simulink model "parcial_2_simulaciones copy"  (R2026b)
settings: Solver=VariableStepAuto  StopTime=20
undefined symbols (not defined in the file): A_LIN, B_LIN, C_LIN, D_LIN, X_INIT
libraries: mpclib x4
settings Model: Creator=santi  LastModifiedBy=ivanm
settings SimscapeCC: SimscapeLogType=all  SimscapeNominalValues="[{\"value\":\"1\",\"unit\":\"A\"},{\"value\":\"1\",\"unit\":\"bar\"},{\"value\":\"1\",\"unit\":\"cm^2\"},{\"value\":\"1\",\"unit\":\"cm^3/s\"},{\"value\":\"1\",\"unit\":\"kJ/kg\"},{\"value\":\"1\",\"unit\":\"kW\"},{\"value\":\"1\",\"unit\":\"l\"},{\"value\":\"1\",\"unit\":\"N\"},{\"value\":\"1\",\"unit\":\"N*m\"},{\"value\":\"1\",\"unit\":\"V\"},{\"value\":\"0.001\",\"unit\":\"Wb\"}]"  SimscapeUseEnergyAccounting=off

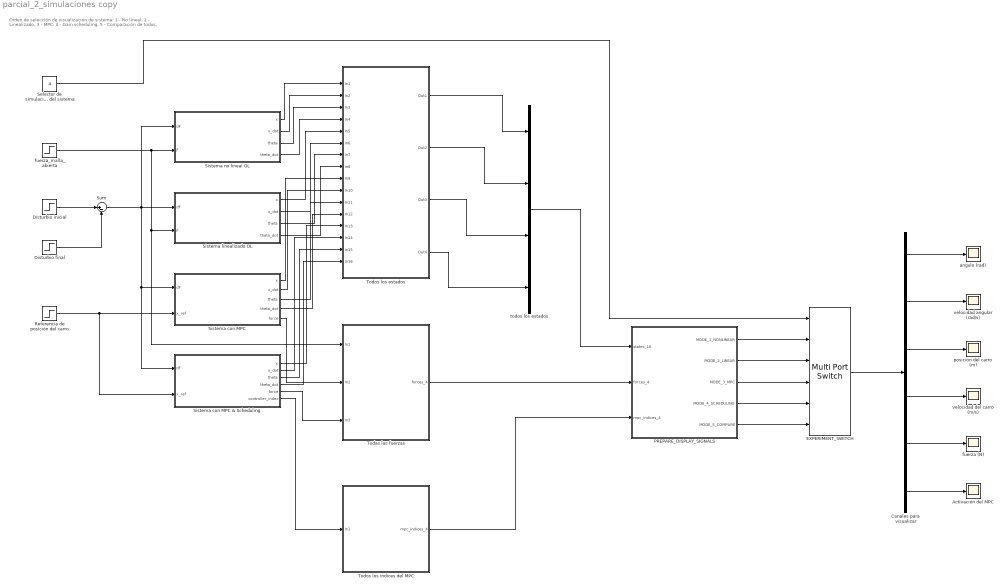
== system parcial_2_simulaciones copy ==
  note: Orden de selección de visualización de sistema:
      |
      | 1 - No lineal.
      | 2 -  Linealizado.
      | 3 - MPC.
      | 4 - Gain scheduling.
      | 5 - Comparación de todos.
  Activación del MPC : Scope
      settings: ActiveDisplayYMinimum=1  ActiveDisplayYMaximum=3  DataLoggingVariableName=ScopeData5
  Canales para visualizar : Demux  Outputs=[4 4 4 4 4 4]
  Disturbio final : Step  Time=4.1  FinalValue=0.05  SampleTime=0
  Disturbio inicial : Step  Time=4  FinalValue=0.05  SampleTime=0
  EXPERIMENT_SWITCH : MultiPortSwitch  Inputs=5  SaturateOnIntegerOverflow=off  InputSameDT=off
  PREPARE_DISPLAY_SIGNALS : Subsystem
  Referencia de posición del carro : Step  FinalValue=0.1  SampleTime=0
  Selector de simulación del sistema : Constant  Value=4
  Sistema con MPC : Subsystem
  Sistema con MPC & Scheduling : Subsystem
  Sistema linealizado OL : Subsystem
  Sistema no lineal OL : Subsystem
  Sum : Sum  Inputs=|+-
  Todas las fuerzas : Subsystem
  Todos los estados : Subsystem
  Todos los indices del MPC : Subsystem
  angulo (rad) : Scope
      settings: ActiveDisplayYMinimum=-0.0688727030292263  ActiveDisplayYMaximum=0.11906082395866187
  fuerza (N) : Scope
      settings: ActiveDisplayYMinimum=-1.8144592130461565  ActiveDisplayYMaximum=0.971895002005476  DataLoggingVariableName=ScopeData4
  fuerza_malla_abierta : Step  Time=0.5  FinalValue=0.05  SampleTime=0
  posición del carro (m) : Scope
      settings: ActiveDisplayYMinimum=-0.040524237311587434  ActiveDisplayYMaximum=0.062688605845198017  DataLoggingVariableName=ScopeData2
  todos los estados : Mux
  velocidad angular (rad/s) : Scope
      settings: ActiveDisplayYMinimum=-0.30702774847885805  ActiveDisplayYMaximum=0.1053556961511582
  velocidad del carro (m/s) : Scope
      settings: ActiveDisplayYMinimum=-0.55827066909262324  ActiveDisplayYMaximum=0.15487434647916765  DataLoggingVariableName=ScopeData3
  wires:
  fuerza_malla_abierta/1 -> Todas las fuerzas/1(In1), Sistema linealizado OL/2(F), Sistema no lineal OL/2(F)
  Disturbio inicial/1 -> Sum/1
  Disturbio final/1 -> Sum/2
  Sum/1 -> Sistema no lineal OL/1(dF), Sistema con MPC/1(dF), Sistema con MPC & Scheduling/1(dF), Sistema linealizado OL/1(dF)
  Referencia de posición del carro/1 -> Sistema con MPC & Scheduling/2(x_ref), Sistema con MPC/2(x_ref)
  Sistema no lineal OL/1(x) -> Todos los estados/1(In1)
  Sistema no lineal OL/2(x_dot) -> Todos los estados/2(In2)
  Sistema no lineal OL/3(theta) -> Todos los estados/3(In3)
  Sistema no lineal OL/4(theta_dot) -> Todos los estados/4(In4)
  Sistema linealizado OL/1(x) -> Todos los estados/5(In5)
  Sistema linealizado OL/2(x_dot) -> Todos los estados/6(In6)
  Sistema linealizado OL/3(theta) -> Todos los estados/7(In7)
  Sistema linealizado OL/4(theta_dot) -> Todos los estados/8(In8)
  Sistema con MPC/1(x) -> Todos los estados/9(In9)
  Sistema con MPC/2(x_dot) -> Todos los estados/10(In10)
  Sistema con MPC/3(theta) -> Todos los estados/11(In11)
  Sistema con MPC/4(theta_dot) -> Todos los estados/12(In12)
  Sistema con MPC & Scheduling/1(x) -> Todos los estados/13(In13)
  Sistema con MPC & Scheduling/2(x_dot) -> Todos los estados/14(In14)
  Sistema con MPC & Scheduling/3(theta) -> Todos los estados/15(In15)
  Sistema con MPC & Scheduling/4(theta_dot) -> Todos los estados/16(In16)
  Sistema con MPC/5(force) -> Todas las fuerzas/2(In2)
  Sistema con MPC & Scheduling/5(force) -> Todas las fuerzas/3(In3)
  Sistema con MPC & Scheduling/6(controller_index) -> Todos los indices del MPC/1(In1)
  PREPARE_DISPLAY_SIGNALS/3(MODE_3_MPC) -> EXPERIMENT_SWITCH/4
  PREPARE_DISPLAY_SIGNALS/4(MODE_4_SCHEDULING) -> EXPERIMENT_SWITCH/5
  PREPARE_DISPLAY_SIGNALS/1(MODE_1_NONLINEAR) -> EXPERIMENT_SWITCH/2
  PREPARE_DISPLAY_SIGNALS/5(MODE_5_COMPARE) -> EXPERIMENT_SWITCH/6
  Todos los estados/1(Out1) -> todos los estados/1
  Todos los estados/2(Out2) -> todos los estados/2
  Todos los estados/3(Out3) -> todos los estados/3
  Todos los estados/4(Out4) -> todos los estados/4
  todos los estados/1 -> PREPARE_DISPLAY_SIGNALS/1(states_16)
  Todas las fuerzas/1(forces_4) -> PREPARE_DISPLAY_SIGNALS/2(forces_4)
  Todos los indices del MPC/1(mpc_indices_4) -> PREPARE_DISPLAY_SIGNALS/3(mpc_indices_4)
  Selector de simulación del sistema/1 -> EXPERIMENT_SWITCH/1
  EXPERIMENT_SWITCH/1 -> Canales para visualizar/1
  Canales para visualizar/1 -> angulo (rad)/1
  Canales para visualizar/2 -> velocidad angular (rad/s)/1
  Canales para visualizar/3 -> posición del carro (m)/1
  Canales para visualizar/4 -> velocidad del carro (m/s)/1
  Canales para visualizar/5 -> fuerza (N)/1
  Canales para visualizar/6 -> Activación del MPC/1
  PREPARE_DISPLAY_SIGNALS/2(MODE_2_LINEAR) -> EXPERIMENT_SWITCH/3

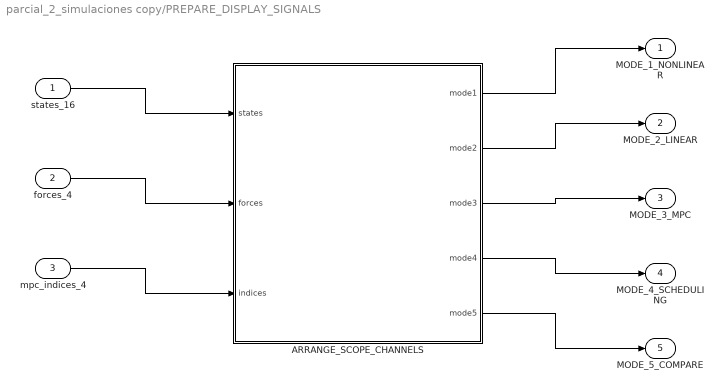
== system parcial_2_simulaciones copy/PREPARE_DISPLAY_SIGNALS ==
  states_16 : Inport
  forces_4 : Inport  Port=2
  mpc_indices_4 : Inport  Port=3
  ARRANGE_SCOPE_CHANNELS : MATLAB Function  TreatAsAtomicUnit=on
  MODE_1_NONLINEAR : Outport
  MODE_2_LINEAR : Outport  Port=2
  MODE_3_MPC : Outport  Port=3
  MODE_4_SCHEDULING : Outport  Port=4
  MODE_5_COMPARE : Outport  Port=5
  wires:
  states_16/1 -> ARRANGE_SCOPE_CHANNELS/1(states)
  forces_4/1 -> ARRANGE_SCOPE_CHANNELS/2(forces)
  mpc_indices_4/1 -> ARRANGE_SCOPE_CHANNELS/3(indices)
  ARRANGE_SCOPE_CHANNELS/1(mode1) -> MODE_1_NONLINEAR/1
  ARRANGE_SCOPE_CHANNELS/2(mode2) -> MODE_2_LINEAR/1
  ARRANGE_SCOPE_CHANNELS/3(mode3) -> MODE_3_MPC/1
  ARRANGE_SCOPE_CHANNELS/4(mode4) -> MODE_4_SCHEDULING/1
  ARRANGE_SCOPE_CHANNELS/5(mode5) -> MODE_5_COMPARE/1

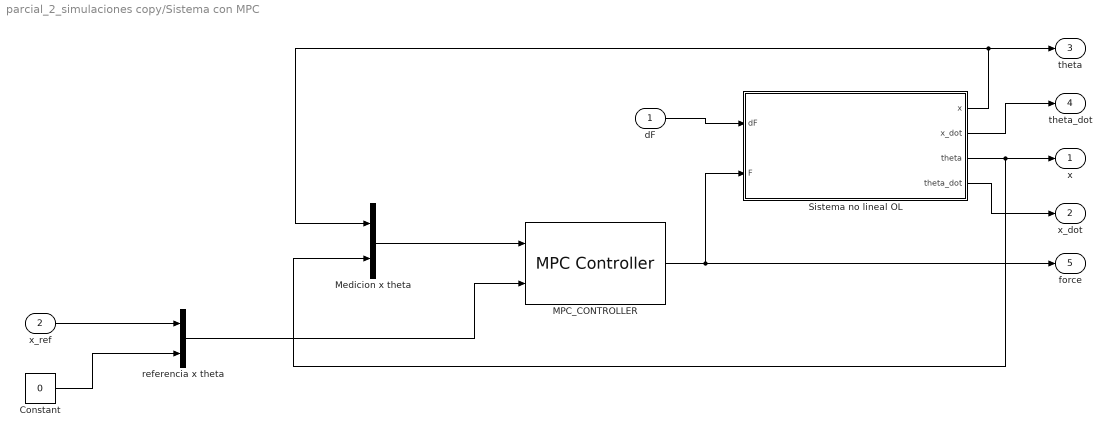
== system parcial_2_simulaciones copy/Sistema con MPC ==
  dF : Inport
  x_ref : Inport  Port=2
  Constant : Constant  Value=0
  MPC_CONTROLLER : mpclib/MPC Controller  SCDEnableBlockLinearizationSpecification=on  mpcobj=mpc_nominal  is_multiple=0  enable_value=0  return_u0=off  updateMPCinCallerWorkspace=on  md_inport=off  mv_inport=off  uref_inport=off  return_cost=off  return_mvseq=off  return_qpstatus=off  return_xseq=off  return_state=off  return_ovseq=off  state_inport=off  umin_inport=off  umax_inport=off  ymin_inport=off  ymax_inport=off  cc_inport=off  ywt_inport=off  uwt_inport=off  duwt_inport=off  rhoeps_inport=off  pm_inport=off  MaximumP=10  HorizonChoice=FixedHorizon  n_ts=0.01  n_p=50  n_mv=1  n_md=0  n_ud=1  n_mo=2  n_uo=0  BlockDataType=double  SampleTimeInherited=off  switch_inport=off
  Medicion x theta : Mux  Inputs=2
  Sistema no lineal OL : Subsystem
  referencia x theta : Mux  Inputs=2
  x : Outport
  x_dot : Outport  Port=2
  theta : Outport  Port=3
  theta_dot : Outport  Port=4
  force : Outport  Port=5
  wires:
  x_ref/1 -> referencia x theta/1
  dF/1 -> Sistema no lineal OL/1(dF)
  MPC_CONTROLLER/1 -> Sistema no lineal OL/2(F), force/1
  Sistema no lineal OL/1(x) -> Medicion x theta/1, theta/1
  Sistema no lineal OL/4(theta_dot) -> x_dot/1
  Sistema no lineal OL/2(x_dot) -> theta_dot/1
  Sistema no lineal OL/3(theta) -> Medicion x theta/2, x/1
  Medicion x theta/1 -> MPC_CONTROLLER/1
  referencia x theta/1 -> MPC_CONTROLLER/2
  Constant/1 -> referencia x theta/2

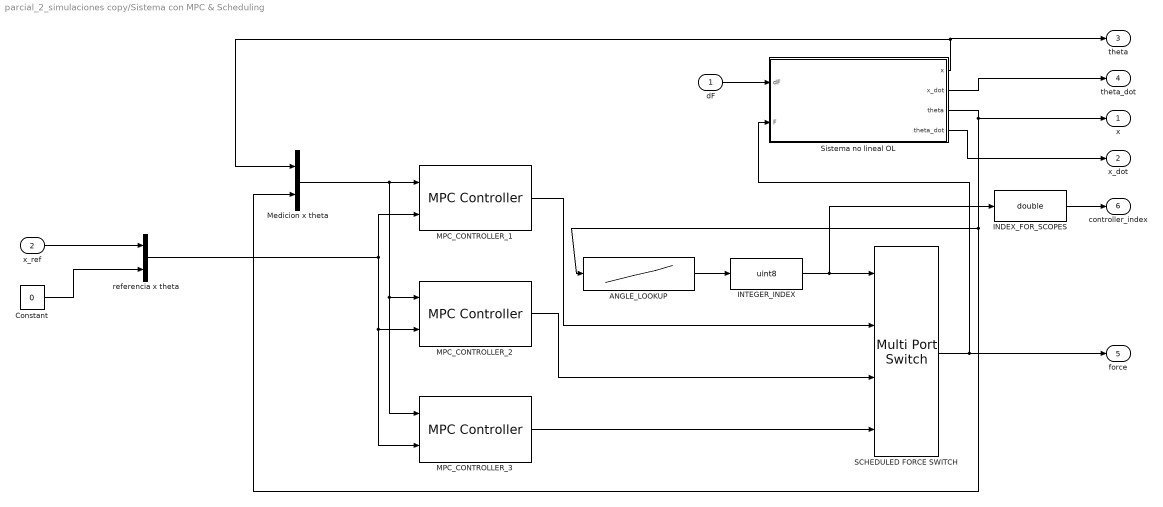
== system parcial_2_simulaciones copy/Sistema con MPC & Scheduling ==
  dF : Inport
  x_ref : Inport  Port=2
  ANGLE_LOOKUP : Lookup_n-D  NumberOfTableDimensions=1  BreakpointsForDimension1=[-4*pi/9 0 4*pi/9]  Table=[1 2 3]  InterpMethod=Nearest  ExtrapMethod=Clip  InternalRulePriority=Speed  RndMeth=Simplest
  Constant : Constant  Value=0
  INDEX_FOR_SCOPES : DataTypeConversion  OutDataTypeStr=double  SaturateOnIntegerOverflow=off  RndMeth=Floor
  INTEGER_INDEX : DataTypeConversion  OutDataTypeStr=uint8  SaturateOnIntegerOverflow=off  RndMeth=Floor
  MPC_CONTROLLER_1 : mpclib/MPC Controller  SCDEnableBlockLinearizationSpecification=on  mpcobj=mpc_nominal  is_multiple=0  enable_value=0  return_u0=off  updateMPCinCallerWorkspace=on  md_inport=off  mv_inport=off  uref_inport=off  return_cost=off  return_mvseq=off  return_qpstatus=off  return_xseq=off  return_state=off  return_ovseq=off  state_inport=off  umin_inport=off  umax_inport=off  ymin_inport=off  ymax_inport=off  cc_inport=off  ywt_inport=off  uwt_inport=off  duwt_inport=off  rhoeps_inport=off  pm_inport=off  MaximumP=10  HorizonChoice=FixedHorizon  n_ts=0.01  n_p=50  n_mv=1  n_md=0  n_ud=1  n_mo=2  n_uo=0  BlockDataType=double  SampleTimeInherited=off  switch_inport=off
  MPC_CONTROLLER_2 : mpclib/MPC Controller  SCDEnableBlockLinearizationSpecification=on  mpcobj=mpc_nominal  is_multiple=0  enable_value=0  return_u0=off  updateMPCinCallerWorkspace=on  md_inport=off  mv_inport=off  uref_inport=off  return_cost=off  return_mvseq=off  return_qpstatus=off  return_xseq=off  return_state=off  return_ovseq=off  state_inport=off  umin_inport=off  umax_inport=off  ymin_inport=off  ymax_inport=off  cc_inport=off  ywt_inport=off  uwt_inport=off  duwt_inport=off  rhoeps_inport=off  pm_inport=off  MaximumP=10  HorizonChoice=FixedHorizon  n_ts=0.01  n_p=50  n_mv=1  n_md=0  n_ud=1  n_mo=2  n_uo=0  BlockDataType=double  SampleTimeInherited=off  switch_inport=off
  MPC_CONTROLLER_3 : mpclib/MPC Controller  SCDEnableBlockLinearizationSpecification=on  mpcobj=mpc_nominal  is_multiple=0  enable_value=0  return_u0=off  updateMPCinCallerWorkspace=on  md_inport=off  mv_inport=off  uref_inport=off  return_cost=off  return_mvseq=off  return_qpstatus=off  return_xseq=off  return_state=off  return_ovseq=off  state_inport=off  umin_inport=off  umax_inport=off  ymin_inport=off  ymax_inport=off  cc_inport=off  ywt_inport=off  uwt_inport=off  duwt_inport=off  rhoeps_inport=off  pm_inport=off  MaximumP=10  HorizonChoice=FixedHorizon  n_ts=0.01  n_p=50  n_mv=1  n_md=0  n_ud=1  n_mo=2  n_uo=0  BlockDataType=double  SampleTimeInherited=off  switch_inport=off
  Medicion x theta : Mux  Inputs=2
  SCHEDULED FORCE SWITCH : MultiPortSwitch  SaturateOnIntegerOverflow=off  InputSameDT=off
  Sistema no lineal OL : Subsystem
  referencia x theta : Mux  Inputs=2
  x : Outport
  x_dot : Outport  Port=2
  theta : Outport  Port=3
  theta_dot : Outport  Port=4
  force : Outport  Port=5
  controller_index : Outport  Port=6
  wires:
  x_ref/1 -> referencia x theta/1
  dF/1 -> Sistema no lineal OL/1(dF)
  MPC_CONTROLLER_1/1 -> SCHEDULED FORCE SWITCH/2
  Sistema no lineal OL/1(x) -> Medicion x theta/1, theta/1
  Sistema no lineal OL/4(theta_dot) -> x_dot/1
  Sistema no lineal OL/2(x_dot) -> theta_dot/1
  Sistema no lineal OL/3(theta) -> Medicion x theta/2, ANGLE_LOOKUP/1, x/1
  Medicion x theta/1 -> MPC_CONTROLLER_1/1, MPC_CONTROLLER_2/1, MPC_CONTROLLER_3/1
  referencia x theta/1 -> MPC_CONTROLLER_2/2, MPC_CONTROLLER_3/2, MPC_CONTROLLER_1/2
  Constant/1 -> referencia x theta/2
  MPC_CONTROLLER_2/1 -> SCHEDULED FORCE SWITCH/3
  MPC_CONTROLLER_3/1 -> SCHEDULED FORCE SWITCH/4
  INTEGER_INDEX/1 -> SCHEDULED FORCE SWITCH/1, INDEX_FOR_SCOPES/1
  ANGLE_LOOKUP/1 -> INTEGER_INDEX/1
  SCHEDULED FORCE SWITCH/1 -> Sistema no lineal OL/2(F), force/1
  INDEX_FOR_SCOPES/1 -> controller_index/1

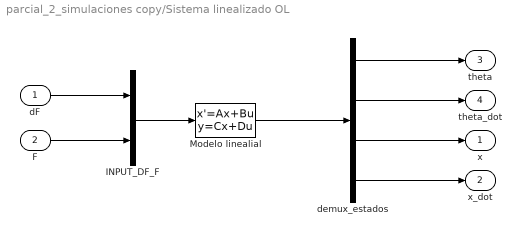
== system parcial_2_simulaciones copy/Sistema linealizado OL ==
  dF : Inport
  F : Inport  Port=2
  INPUT_DF_F : Mux  Inputs=2
  Modelo linealial : StateSpace  A=A_LIN  B=B_LIN(:,[2 1])  C=C_LIN  D=D_LIN(:,[2 1])  InitialCondition=X_INIT
  demux_estados : Demux
  x : Outport
  x_dot : Outport  Port=2
  theta : Outport  Port=3
  theta_dot : Outport  Port=4
  wires:
  dF/1 -> INPUT_DF_F/1
  F/1 -> INPUT_DF_F/2
  INPUT_DF_F/1 -> Modelo linealial/1
  Modelo linealial/1 -> demux_estados/1
  demux_estados/2 -> theta_dot/1
  demux_estados/3 -> x/1
  demux_estados/4 -> x_dot/1
  demux_estados/1 -> theta/1

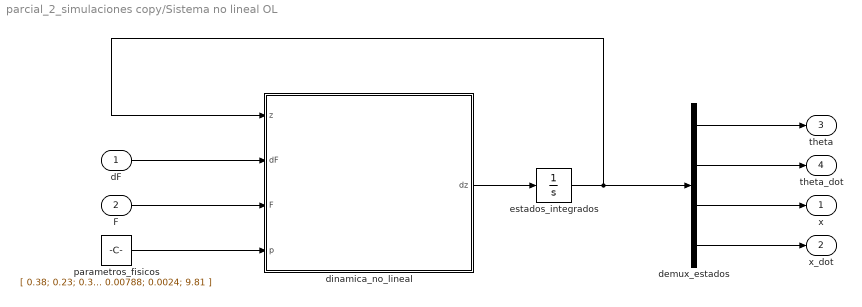
== system parcial_2_simulaciones copy/Sistema no lineal OL ==
  dF : Inport
  F : Inport  Port=2
  demux_estados : Demux
  dinamica_no_lineal : MATLAB Function  TreatAsAtomicUnit=on
  estados_integrados : Integrator  InitialCondition=X_INIT
  parametros_fisicos : Constant  Value=[ 0.38; 0.23; 0.3302; 0.00788; 0.0024; 9.81 ]
  x : Outport
  x_dot : Outport  Port=2
  theta : Outport  Port=3
  theta_dot : Outport  Port=4
  wires:
  demux_estados/2 -> theta_dot/1
  parametros_fisicos/1 -> dinamica_no_lineal/4(p)
  demux_estados/1 -> theta/1
  estados_integrados/1 -> dinamica_no_lineal/1(z), demux_estados/1
  dinamica_no_lineal/1(dz) -> estados_integrados/1
  demux_estados/4 -> x_dot/1
  F/1 -> dinamica_no_lineal/3(F)
  dF/1 -> dinamica_no_lineal/2(dF)
  demux_estados/3 -> x/1

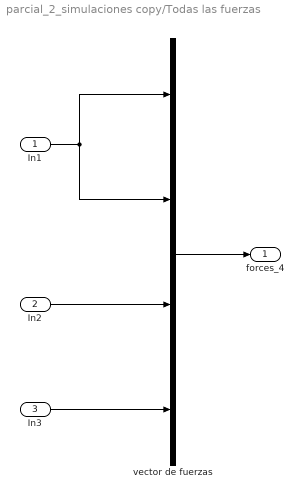
== system parcial_2_simulaciones copy/Todas las fuerzas ==
  In1 : Inport
  In2 : Inport  Port=2
  In3 : Inport  Port=3
  vector de fuerzas : Mux
  forces_4 : Outport
  wires:
  vector de fuerzas/1 -> forces_4/1
  In2/1 -> vector de fuerzas/3
  In1/1 -> vector de fuerzas/2, vector de fuerzas/1
  In3/1 -> vector de fuerzas/4

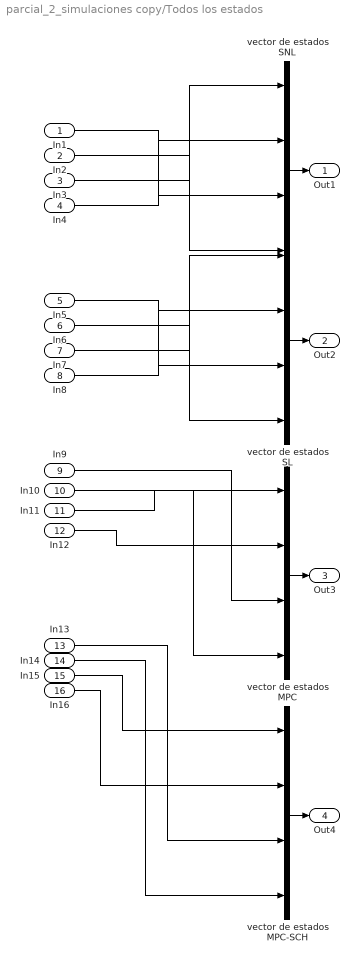
== system parcial_2_simulaciones copy/Todos los estados ==
  In1 : Inport
  In2 : Inport  Port=2
  In3 : Inport  Port=3
  In4 : Inport  Port=4
  In5 : Inport  Port=5
  In6 : Inport  Port=6
  In7 : Inport  Port=7
  In8 : Inport  Port=8
  In9 : Inport  Port=9
  In10 : Inport  Port=10
  In11 : Inport  Port=11
  In12 : Inport  Port=12
  In13 : Inport  Port=13
  In14 : Inport  Port=14
  In15 : Inport  Port=15
  In16 : Inport  Port=16
  vector de estados MPC : Mux
  vector de estados MPC-SCH : Mux
  vector de estados SL : Mux
  "vector de estados SNL " : Mux
  Out1 : Outport
  Out2 : Outport  Port=2
  Out3 : Outport  Port=3
  Out4 : Outport  Port=4
  wires:
  vector de estados MPC-SCH/1 -> Out4/1
  In4/1 -> "vector de estados SNL "/2
  In1/1 -> "vector de estados SNL "/3
  "vector de estados SNL "/1 -> Out1/1
  In2/1 -> "vector de estados SNL "/4
  In7/1 -> vector de estados SL/1
  In3/1 -> "vector de estados SNL "/1
  In12/1 -> vector de estados MPC/2
  vector de estados SL/1 -> Out2/1
  In6/1 -> vector de estados SL/4
  In5/1 -> vector de estados SL/3
  In9/1 -> vector de estados MPC/3
  In8/1 -> vector de estados SL/2
  In10/1 -> vector de estados MPC/4
  In11/1 -> vector de estados MPC/1
  vector de estados MPC/1 -> Out3/1
  In13/1 -> vector de estados MPC-SCH/3
  In14/1 -> vector de estados MPC-SCH/4
  In15/1 -> vector de estados MPC-SCH/1
  In16/1 -> vector de estados MPC-SCH/2

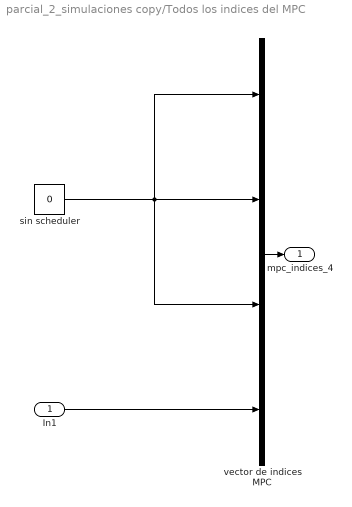
== system parcial_2_simulaciones copy/Todos los indices del MPC ==
  In1 : Inport
  sin scheduler : Constant  Value=0
  vector de indices MPC : Mux
  mpc_indices_4 : Outport
  wires:
  sin scheduler/1 -> vector de indices MPC/1, vector de indices MPC/2, vector de indices MPC/3
  vector de indices MPC/1 -> mpc_indices_4/1
  In1/1 -> vector de indices MPC/4

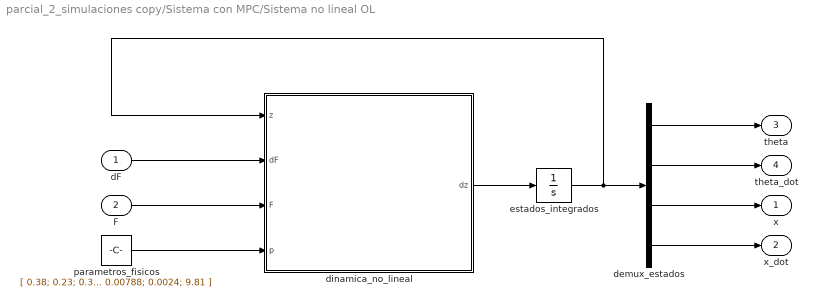
== system parcial_2_simulaciones copy/Sistema con MPC/Sistema no lineal OL ==
  dF : Inport
  F : Inport  Port=2
  demux_estados : Demux
  dinamica_no_lineal : MATLAB Function  TreatAsAtomicUnit=on
  estados_integrados : Integrator  InitialCondition=X_INIT
  parametros_fisicos : Constant  Value=[ 0.38; 0.23; 0.3302; 0.00788; 0.0024; 9.81 ]
  x : Outport
  x_dot : Outport  Port=2
  theta : Outport  Port=3
  theta_dot : Outport  Port=4
  wires:
  parametros_fisicos/1 -> dinamica_no_lineal/4(p)
  dinamica_no_lineal/1(dz) -> estados_integrados/1
  F/1 -> dinamica_no_lineal/3(F)
  dF/1 -> dinamica_no_lineal/2(dF)
  estados_integrados/1 -> demux_estados/1, dinamica_no_lineal/1(z)
  demux_estados/2 -> theta_dot/1
  demux_estados/3 -> x/1
  demux_estados/4 -> x_dot/1
  demux_estados/1 -> theta/1

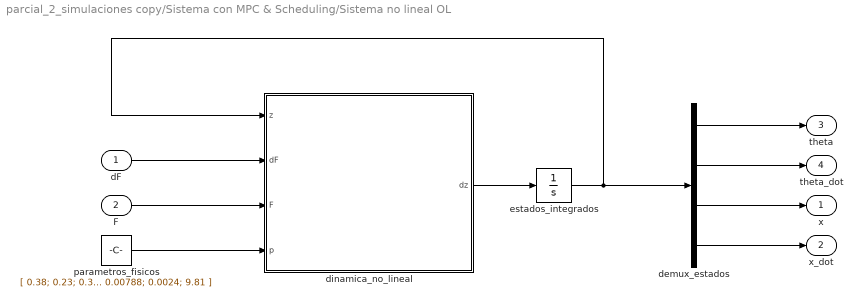
== system parcial_2_simulaciones copy/Sistema con MPC & Scheduling/Sistema no lineal OL ==
  dF : Inport
  F : Inport  Port=2
  demux_estados : Demux
  dinamica_no_lineal : MATLAB Function  TreatAsAtomicUnit=on
  estados_integrados : Integrator  InitialCondition=X_INIT
  parametros_fisicos : Constant  Value=[ 0.38; 0.23; 0.3302; 0.00788; 0.0024; 9.81 ]
  x : Outport
  x_dot : Outport  Port=2
  theta : Outport  Port=3
  theta_dot : Outport  Port=4
  wires:
  demux_estados/2 -> theta_dot/1
  parametros_fisicos/1 -> dinamica_no_lineal/4(p)
  demux_estados/1 -> theta/1
  estados_integrados/1 -> dinamica_no_lineal/1(z), demux_estados/1
  dinamica_no_lineal/1(dz) -> estados_integrados/1
  demux_estados/4 -> x_dot/1
  F/1 -> dinamica_no_lineal/3(F)
  dF/1 -> dinamica_no_lineal/2(dF)
  demux_estados/3 -> x/1

== matlab function parcial_2_simulaciones copy/Sistema con MPC/Sistema no lineal OL/dinamica_no_lineal ==
  data: z input; dz output; dF input; F input; p input
function dz = cartpole_dynamics(z,dF,F,p)
%#codegen
theta = z(1);
omega = z(2);
v = z(4);
M = p(1); m = p(2); l = p(3);
I = p(4); b = p(5); g = p(6);
c = cos(theta); si = sin(theta);
rhs1 = F-dF-b*v-m*l*si*omega^2;
rhs2 = dF*l*c+m*g*l*si;
den = (M+m)*(I+m*l^2)-(m*l*c)^2;
xdd = ((I+m*l^2)*rhs1+m*l*c*rhs2)/den;
tdd = (m*l*c*rhs1+(M+m)*rhs2)/den;
dz = [omega;tdd;v;xdd];
end

== matlab function parcial_2_simulaciones copy/Sistema no lineal OL/dinamica_no_lineal ==
  data: z input; dz output; dF input; F input; p input
function dz = cartpole_dynamics(z,dF,F,p)
%#codegen
theta = z(1);
omega = z(2);
v = z(4);
M = p(1); m = p(2); l = p(3);
I = p(4); b = p(5); g = p(6);
c = cos(theta); si = sin(theta);
rhs1 = F-dF-b*v-m*l*si*omega^2;
rhs2 = dF*l*c+m*g*l*si;
den = (M+m)*(I+m*l^2)-(m*l*c)^2;
xdd = ((I+m*l^2)*rhs1+m*l*c*rhs2)/den;
tdd = (m*l*c*rhs1+(M+m)*rhs2)/den;
dz = [omega;tdd;v;xdd];
end

== matlab function parcial_2_simulaciones copy/Sistema con MPC & Scheduling/Sistema no lineal OL/dinamica_no_lineal ==
  data: z input; dz output; dF input; F input; p input
function dz = cartpole_dynamics(z,dF,F,p)
%#codegen
theta = z(1);
omega = z(2);
v = z(4);
M = p(1); m = p(2); l = p(3);
I = p(4); b = p(5); g = p(6);
c = cos(theta); si = sin(theta);
rhs1 = F-dF-b*v-m*l*si*omega^2;
rhs2 = dF*l*c+m*g*l*si;
den = (M+m)*(I+m*l^2)-(m*l*c)^2;
xdd = ((I+m*l^2)*rhs1+m*l*c*rhs2)/den;
tdd = (m*l*c*rhs1+(M+m)*rhs2)/den;
dz = [omega;tdd;v;xdd];
end

== matlab function parcial_2_simulaciones copy/PREPARE_DISPLAY_SIGNALS/ARRANGE_SCOPE_CHANNELS ==
  data: states input; mode1 output; forces input; indices input; mode2 output; mode3 output; mode4 output; mode5 output
function [mode1,mode2,mode3,mode4,mode5] = arrange_views(states,forces,indices)
%#codegen
views = nan(24,5);
for k = 1:4
    offset = 4*(k-1);
    signals = [states(offset+1);states(offset+2);states(offset+3);states(offset+4);forces(k);indices(k)];
    for j = 1:6
        row = 4*(j-1)+k;
        views(row,k) = signals(j);
        views(row,5) = signals(j);
    end
end
mode1 = views(:,1);
mode2 = views(:,2);
mode3 = views(:,3);
mode4 = views(:,4);
mode5 = views(:,5);
end
